simulink model "Modellering"  (R2026a)
settings: Solver=VariableStepAuto  StopTime=24*T_time  AbsTol=1e-3
values from neighbouring files (symbols this model uses):
  E_batt_Wh = 1e3    (= 1000)    [Solcelle_KW_PR_KWP.m]
  pf_fabrik = 0.85    [Last_fra_fabrik_blokkode.m]
  T_time = 0.2    [Solcelle_KW_PR_KWP.m]
libraries: ee_lib x24, nesl_utility x23, eeSinGeneratorThreePhase x3, fl_lib x2
settings Model: Creator=Tjalf  LastModifiedBy=Tjalf
settings DebuggingCC: SymbolicDimsDataTypeCodeGenerationDiagnostic=none

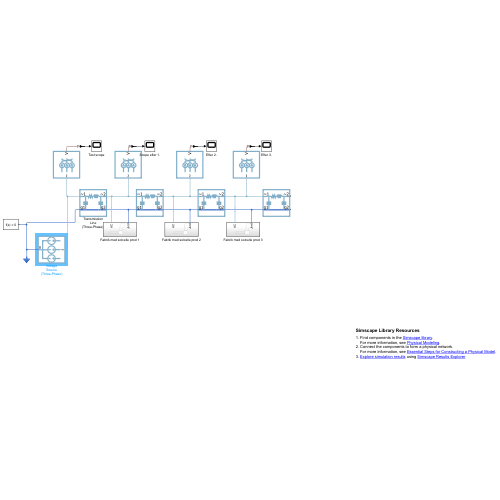
[thumbnail: Simulink's stored preview of the top-level diagram]
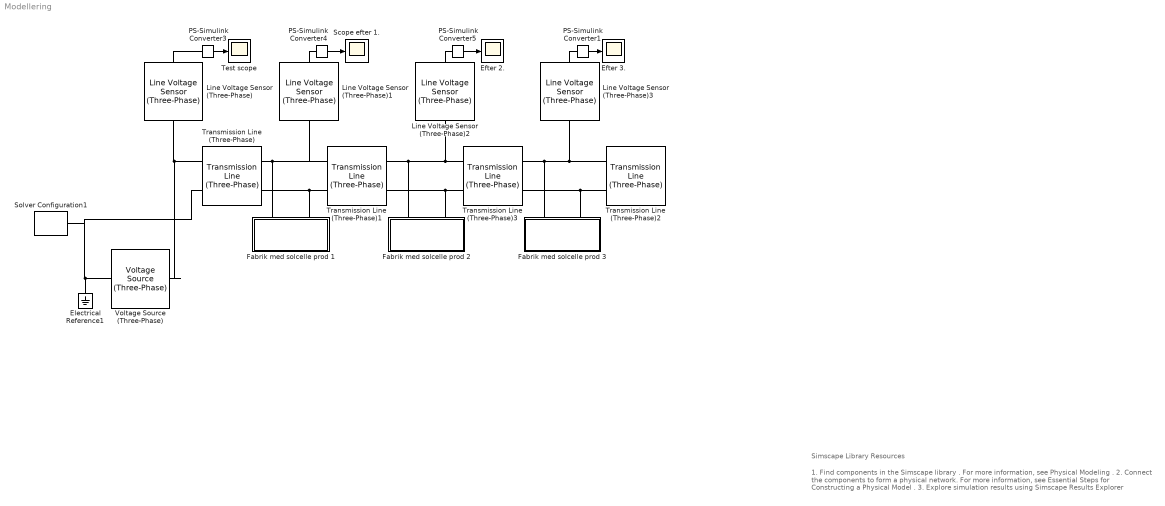
== system Modellering ==
  note: 1. Find components in the Simscape library .
      | For more information, see Physical Modeling .
      | 2. Connect the components to form a physical network.
      | For more information, see Essential Steps for Constructing a Physical Model .
      | 3. Explore simulation results using Simscape Results Explorer
  note: Simscape Library Resources
  Efter 2. : Scope
      settings: ActiveDisplayYMinimum=-525.7657436259899  ActiveDisplayYMaximum=512.09070122953233  DataLoggingVariableName=ScopeData5
  Efter 3. : Scope
      settings: ActiveDisplayYMinimum=-108.97469280207605  ActiveDisplayYMaximum=205.85166313411651  DataLoggingVariableName=ScopeData2
  Electrical Reference1 : fl_lib/Electrical/Electrical Elements/Electrical Reference
  Fabrik med solcelle prod 1 : Subsystem
      settings: PortSchema="{\"entries\":[{\"content\":{\"sides\":[{\"content\":{},\"type\":\"ConnectorPlacement.EquallySpacedRectSide\",\"uuid\":\"8903bc28-abed-4d25-a485-866d339a2aaa\"},{\"content\":{\"side\":\"RIGHT\"},\"type\":\"ConnectorPlacement.EquallySpacedRectSide\",\"uuid\":\"5b54d37e-ff1f-4c27-bd8c-71a5161d98d9\"},{\"content\":{\"connectorIds\":[\"LConn1\",\"LConn2\"],\"side\":\"TOP\"},\"type\":\"ConnectorPlacement.EquallySpacedRectSide\",\"uuid\":\"1a79fc57-00bb-46c3-a083-8bac977ee0cf\"},{\"content\":{\"side\":\"BOTTOM\"},\"type\":\"ConnectorPlacement.EquallySpacedRectSide\",\"uuid\":\"fed7dcc3-d9d7-4755-8d81-a67162f2978b\"}]},\"type\":\"ConnectorPlacement.EquallySpacedConnector\",\"uuid\":\"4f69986a-bdbb-438c-8339-f1c9bb70dacd\"}],\"packageUris\":[\"http://schema.mathworks.com/mf0/Connector/R2020b\"],\"version\":\"1.0\"}"
  Fabrik med solcelle prod 2 : Subsystem
      settings: PortSchema="{\"entries\":[{\"content\":{\"sides\":[{\"content\":{},\"type\":\"ConnectorPlacement.EquallySpacedRectSide\",\"uuid\":\"8903bc28-abed-4d25-a485-866d339a2aaa\"},{\"content\":{\"side\":\"RIGHT\"},\"type\":\"ConnectorPlacement.EquallySpacedRectSide\",\"uuid\":\"5b54d37e-ff1f-4c27-bd8c-71a5161d98d9\"},{\"content\":{\"connectorIds\":[\"LConn1\",\"LConn2\"],\"side\":\"TOP\"},\"type\":\"ConnectorPlacement.EquallySpacedRectSide\",\"uuid\":\"1a79fc57-00bb-46c3-a083-8bac977ee0cf\"},{\"content\":{\"side\":\"BOTTOM\"},\"type\":\"ConnectorPlacement.EquallySpacedRectSide\",\"uuid\":\"fed7dcc3-d9d7-4755-8d81-a67162f2978b\"}]},\"type\":\"ConnectorPlacement.EquallySpacedConnector\",\"uuid\":\"4f69986a-bdbb-438c-8339-f1c9bb70dacd\"}],\"packageUris\":[\"http://schema.mathworks.com/mf0/Connector/R2020b\"],\"version\":\"1.0\"}"
  Fabrik med solcelle prod 3 : Subsystem
      settings: PortSchema="{\"entries\":[{\"content\":{\"sides\":[{\"content\":{},\"type\":\"ConnectorPlacement.EquallySpacedRectSide\",\"uuid\":\"8903bc28-abed-4d25-a485-866d339a2aaa\"},{\"content\":{\"side\":\"RIGHT\"},\"type\":\"ConnectorPlacement.EquallySpacedRectSide\",\"uuid\":\"5b54d37e-ff1f-4c27-bd8c-71a5161d98d9\"},{\"content\":{\"connectorIds\":[\"LConn1\",\"LConn2\"],\"side\":\"TOP\"},\"type\":\"ConnectorPlacement.EquallySpacedRectSide\",\"uuid\":\"1a79fc57-00bb-46c3-a083-8bac977ee0cf\"},{\"content\":{\"side\":\"BOTTOM\"},\"type\":\"ConnectorPlacement.EquallySpacedRectSide\",\"uuid\":\"fed7dcc3-d9d7-4755-8d81-a67162f2978b\"}]},\"type\":\"ConnectorPlacement.EquallySpacedConnector\",\"uuid\":\"4f69986a-bdbb-438c-8339-f1c9bb70dacd\"}],\"packageUris\":[\"http://schema.mathworks.com/mf0/Connector/R2020b\"],\"version\":\"1.0\"}"
  Line Voltage Sensor (Three-Phase){,1..3} (4 alike) : ee_lib/Sensors & Transducers/Line Voltage Sensor (Three-Phase)  port_option=ee.enum.threePhasePort.composite
  PS-Simulink Converter{1,3..5} (4 alike) : nesl_utility/PS-Simulink Converter  PhysicalDomain=network_engine_domain  SubClassName=ps_output  LeftPortType=input  RightPortType=output  PseudoPeriodic=off  Frequencies=[]  VectorFormat=inherit  Unit=V  AffineConversion=off
  Scope efter 1. : Scope
      settings: ActiveDisplayYMinimum=-808.59258984260134  ActiveDisplayYMaximum=1226.7327895966071  DataLoggingVariableName=ScopeData4
  Solver Configuration1 : nesl_utility/Solver Configuration  PhysicalDomain=network_engine_domain  SubClassName=solver  LeftPortType=input  RightPortType=generic  Tones=[]  Harmonics=[]  SimulateNoise=off  Profile=off  UseLocalSampling=off  EnableSwitchedLinearOptims=on  FrequencyDomain=off  UseCCode=off  RelTol=0.001  AbsTol=0.001  MinStep=1e-09  ToWorkspace=off  RevertToSquareIcSolve=off  NumHomotopyIterations=100  PhasorMode=off  PhasorModeNumHarmonics=1  ConsistencySolver=NEWTON_XTOL_AFTER_FTOL  CanonicalOrdering=CANONICAL  OptimizeIntermediates=OPTIMIZED  IndexReductionMethod=DerivativeReplacement  DoDC=off  ResidualTolerance=1e-09  ConsistencyTolSource=GLOBAL  ConsistencyAbsTol=0.001  ConsistencyRelTol=0.001  ConsistencyTolFactor=0.001  UseLocalSolver=on  LocalSolverChoice=NE_BACKWARD_EULER_ADVANCER  ResolveIndetEquations=on  FunctionEvalNumThread=1  LocalSolverSampleTime=1e-4  DoFixedCost=off  MaxNonlinIter=3  MaxModeIter=2  ComputeImpulses=off  ImpulseIterations=2  LinearAlgebra=auto  LinearAlgebraNumThread=0  EquationFormulation=NE_TIME_EF  DelaysMemoryBudget=1024  AutomaticFiltering=on  FilteringTimeConstant=0.001  PartitionStorageMethod=AS_NEEDED  PartitionMemoryBudget=1024  PartitionMethod=ROBUST  MultibodyUseLocalSolver=off  MultibodyLocalSolverChoice=ODE1  MultibodyLocalSolverSampleTime=0.001
  Test scope : Scope
      settings: ActiveDisplayYMinimum=-725.330758823431  ActiveDisplayYMaximum=222.55952159059962  DataLoggingVariableName=ScopeData3
  "Transmission Line (Three-Phase) " : ee_lib/Passive/Lines/Transmission Line (Three-Phase)  port_option=ee.enum.threePhasePort.composite  length=0.4 km  freq=50 Hz  prm=ee.enum.lines.parameterization3ph.physicalLineParam  R=0.34 Ohm/km  Rm=0 Ohm/km  L=0.5 mH/km  M=0.1 mH/km  Cl=0.3 uF/km  Cg=0.1 uF/km  Rpos=0.01 Ohm/km  Rzero=0.04 Ohm/km  Lpos=0.4 mH/km  Lzero=0.7 mH/km  Cpos=1 uF/km  Czero=0.1 uF/km  ModelTwoSections=ee.enum.enable.no  N=1  InterfacePosition=0.5 km  N1sec=1  N2sec=1  Access_ground=ee.enum.enable.no  R_parasitic=1e-6 Ohm  G_parasitic=1e-6 1/Ohm
  Transmission Line (Three-Phase)1 : ee_lib/Passive/Lines/Transmission Line (Three-Phase)  port_option=ee.enum.threePhasePort.composite  length=0.2 km  freq=50 Hz  prm=ee.enum.lines.parameterization3ph.physicalLineParam  R=0.34 Ohm/km  Rm=0 Ohm/km  L=0.5 mH/km  M=0.1 mH/km  Cl=0.3 uF/km  Cg=0.1 uF/km  Rpos=0.01 Ohm/km  Rzero=0.04 Ohm/km  Lpos=0.4 mH/km  Lzero=0.7 mH/km  Cpos=1 uF/km  Czero=0.1 uF/km  ModelTwoSections=ee.enum.enable.no  N=1  InterfacePosition=0.5 km  N1sec=1  N2sec=1  Access_ground=ee.enum.enable.no  R_parasitic=1e-6 Ohm  G_parasitic=1e-6 1/Ohm
  Transmission Line (Three-Phase)2 : ee_lib/Passive/Lines/Transmission Line (Three-Phase)  port_option=ee.enum.threePhasePort.composite  length=0.3 km  freq=50 Hz  prm=ee.enum.lines.parameterization3ph.physicalLineParam  R=0.34 Ohm/km  Rm=0 Ohm/km  L=0.5 mH/km  M=0.1 mH/km  Cl=0.3 uF/km  Cg=0.1 uF/km  Rpos=0.01 Ohm/km  Rzero=0.04 Ohm/km  Lpos=0.4 mH/km  Lzero=0.7 mH/km  Cpos=1 uF/km  Czero=0.1 uF/km  ModelTwoSections=ee.enum.enable.no  N=1  InterfacePosition=0.5 km  N1sec=1  N2sec=1  Access_ground=ee.enum.enable.no  R_parasitic=1e-6 Ohm  G_parasitic=1e-6 1/Ohm
  Transmission Line (Three-Phase)3 : ee_lib/Passive/Lines/Transmission Line (Three-Phase)  port_option=ee.enum.threePhasePort.composite  length=0.3 km  freq=50 Hz  prm=ee.enum.lines.parameterization3ph.physicalLineParam  R=0.34 Ohm/km  Rm=0 Ohm/km  L=0.5 mH/km  M=0.1 mH/km  Cl=0.3 uF/km  Cg=0.1 uF/km  Rpos=0.01 Ohm/km  Rzero=0.04 Ohm/km  Lpos=0.4 mH/km  Lzero=0.7 mH/km  Cpos=1 uF/km  Czero=0.1 uF/km  ModelTwoSections=ee.enum.enable.no  N=1  InterfacePosition=0.5 km  N1sec=1  N2sec=1  Access_ground=ee.enum.enable.no  R_parasitic=1e-6 Ohm  G_parasitic=1e-6 1/Ohm
  Voltage Source (Three-Phase) : ee_lib/Sources/Voltage Source (Three-Phase)  vline_rms=400 V  shift=0 deg  freq=50 Hz  impedance_option=1  SShortCircuit=1e9 A*V  XR=15  R=0.01 Ohm  L=3.97e-4 H  harmonic_option=0  harmonic_orders=[5, 7, 11, 13]  harmonic_ratios=[.1, .1, .1, .1]  G_parasitic=0 1/Ohm  I_specify=off  I_priority=None  I=[0, 0, 0] A  I_nominal_specify=off  I_nominal_value=1  I_nominal_unit=A
  wires:
  PS-Simulink Converter3/1 -> Test scope/1
  PS-Simulink Converter4/1 -> Scope efter 1./1
  PS-Simulink Converter5/1 -> Efter 2./1
  PS-Simulink Converter1/1 -> Efter 3./1
  connections:
  Electrical Reference1/LConn1 -- "Transmission Line (Three-Phase) "/LConn2 -- Solver Configuration1/RConn1 -- Voltage Source (Three-Phase)/LConn1
  Voltage Source (Three-Phase)/RConn1 -- Line Voltage Sensor (Three-Phase)/LConn1 -- "Transmission Line (Three-Phase) "/LConn1
  Transmission Line (Three-Phase)3/LConn1 -- Fabrik med solcelle prod 2/LConn1 -- Transmission Line (Three-Phase)1/RConn1 -- Line Voltage Sensor (Three-Phase)2/LConn1
  Transmission Line (Three-Phase)3/LConn2 -- Fabrik med solcelle prod 2/LConn2 -- Transmission Line (Three-Phase)1/RConn2
  Transmission Line (Three-Phase)1/LConn2 -- Fabrik med solcelle prod 1/LConn2 -- "Transmission Line (Three-Phase) "/RConn2
  "Transmission Line (Three-Phase) "/RConn1 -- Transmission Line (Three-Phase)1/LConn1 -- Line Voltage Sensor (Three-Phase)1/LConn1 -- Fabrik med solcelle prod 1/LConn1
  Line Voltage Sensor (Three-Phase)/RConn1 -- PS-Simulink Converter3/LConn1
  Line Voltage Sensor (Three-Phase)1/RConn1 -- PS-Simulink Converter4/LConn1
  Line Voltage Sensor (Three-Phase)2/RConn1 -- PS-Simulink Converter5/LConn1
  Line Voltage Sensor (Three-Phase)3/RConn1 -- PS-Simulink Converter1/LConn1
  Line Voltage Sensor (Three-Phase)3/LConn1 -- Fabrik med solcelle prod 3/LConn1 -- Transmission Line (Three-Phase)3/RConn1 -- Transmission Line (Three-Phase)2/LConn1
  Transmission Line (Three-Phase)2/LConn2 -- Fabrik med solcelle prod 3/LConn2 -- Transmission Line (Three-Phase)3/RConn2

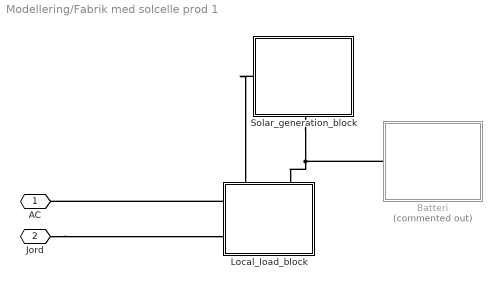
== system Modellering/Fabrik med solcelle prod 1 ==
  Batteri : Subsystem  Commented=on
  Local_load_block : Subsystem
      settings: PortSchema="{\"entries\":[{\"content\":{\"sides\":[{\"content\":{\"connectorIds\":[\"LConn1\",\"LConn2\"]},\"type\":\"ConnectorPlacement.EquallySpacedRectSide\",\"uuid\":\"b9fbc9ff-ac4f-4b90-979a-9a6eda85b56b\"},{\"content\":{\"side\":\"RIGHT\"},\"type\":\"ConnectorPlacement.EquallySpacedRectSide\",\"uuid\":\"0bc181a9-ce47-4155-858d-d096cf0eda13\"},{\"content\":{\"connectorIds\":[\"LConn3\",\"LConn4\"],\"side\":\"TOP\"},\"type\":\"ConnectorPlacement.EquallySpacedRectSide\",\"uuid\":\"c62c2ae1-dcbf-4404-92e0-79f349a5ed39\"}]},\"type\":\"ConnectorPlacement.EquallySpacedConnector\",\"uuid\":\"35e445ba-d9d4-4891-abed-fc367708c4b2\"}],\"packageUris\":[\"http://schema.mathworks.com/mf0/Connector/R2020b\"],\"version\":\"1.0\"}"
  Solar_generation_block : Subsystem
      settings: PortSchema="{\"entries\":[{\"content\":{\"sides\":[{\"content\":{\"connectorIds\":[\"LConn1\"]},\"type\":\"ConnectorPlacement.EquallySpacedRectSide\",\"uuid\":\"cbc424fc-8eab-49e5-bd35-99b901f58cde\"},{\"content\":{\"side\":\"RIGHT\"},\"type\":\"ConnectorPlacement.EquallySpacedRectSide\",\"uuid\":\"42c77621-fd98-407f-9927-3f3ead5ecc38\"},{\"content\":{\"side\":\"TOP\"},\"type\":\"ConnectorPlacement.EquallySpacedRectSide\",\"uuid\":\"f218016a-264e-4591-beac-7ee07d8c289f\"},{\"content\":{\"connectorIds\":[\"RConn1\"],\"side\":\"BOTTOM\"},\"type\":\"ConnectorPlacement.EquallySpacedRectSide\",\"uuid\":\"65d2543d-d490-4083-b53c-51918d15ba9f\"}]},\"type\":\"ConnectorPlacement.EquallySpacedConnector\",\"uuid\":\"55afaa4f-6643-4b7e-8511-738cdc79d4c6\"}],\"packageUris\":[\"http://schema.mathworks.com/mf0/Connector/R2020b\"],\"version\":\"1.0\"}"
  AC : PMIOPort  Side=Left
  Jord : PMIOPort  Port=2  Side=Left
  connections:
  Local_load_block/LConn1 -- AC/RConn1
  Jord/RConn1 -- Local_load_block/LConn2
  Solar_generation_block/LConn1 -- Local_load_block/LConn3
  Solar_generation_block/RConn1 -- Batteri/LConn1 -- Local_load_block/LConn4

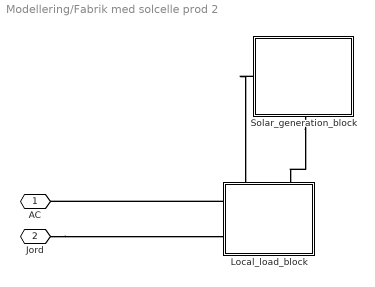
== system Modellering/Fabrik med solcelle prod 2 ==
  Local_load_block : Subsystem
      settings: PortSchema="{\"entries\":[{\"content\":{\"sides\":[{\"content\":{\"connectorIds\":[\"LConn1\",\"LConn2\"]},\"type\":\"ConnectorPlacement.EquallySpacedRectSide\",\"uuid\":\"b9fbc9ff-ac4f-4b90-979a-9a6eda85b56b\"},{\"content\":{\"side\":\"RIGHT\"},\"type\":\"ConnectorPlacement.EquallySpacedRectSide\",\"uuid\":\"0bc181a9-ce47-4155-858d-d096cf0eda13\"},{\"content\":{\"connectorIds\":[\"LConn3\",\"LConn4\"],\"side\":\"TOP\"},\"type\":\"ConnectorPlacement.EquallySpacedRectSide\",\"uuid\":\"c62c2ae1-dcbf-4404-92e0-79f349a5ed39\"}]},\"type\":\"ConnectorPlacement.EquallySpacedConnector\",\"uuid\":\"35e445ba-d9d4-4891-abed-fc367708c4b2\"}],\"packageUris\":[\"http://schema.mathworks.com/mf0/Connector/R2020b\"],\"version\":\"1.0\"}"
  Solar_generation_block : Subsystem
      settings: PortSchema="{\"entries\":[{\"content\":{\"sides\":[{\"content\":{\"connectorIds\":[\"LConn1\"]},\"type\":\"ConnectorPlacement.EquallySpacedRectSide\",\"uuid\":\"cbc424fc-8eab-49e5-bd35-99b901f58cde\"},{\"content\":{\"side\":\"RIGHT\"},\"type\":\"ConnectorPlacement.EquallySpacedRectSide\",\"uuid\":\"42c77621-fd98-407f-9927-3f3ead5ecc38\"},{\"content\":{\"side\":\"TOP\"},\"type\":\"ConnectorPlacement.EquallySpacedRectSide\",\"uuid\":\"f218016a-264e-4591-beac-7ee07d8c289f\"},{\"content\":{\"connectorIds\":[\"RConn1\"],\"side\":\"BOTTOM\"},\"type\":\"ConnectorPlacement.EquallySpacedRectSide\",\"uuid\":\"65d2543d-d490-4083-b53c-51918d15ba9f\"}]},\"type\":\"ConnectorPlacement.EquallySpacedConnector\",\"uuid\":\"55afaa4f-6643-4b7e-8511-738cdc79d4c6\"}],\"packageUris\":[\"http://schema.mathworks.com/mf0/Connector/R2020b\"],\"version\":\"1.0\"}"
  AC : PMIOPort  Side=Left
  Jord : PMIOPort  Port=2  Side=Left
  connections:
  Solar_generation_block/RConn1 -- Local_load_block/LConn4
  Solar_generation_block/LConn1 -- Local_load_block/LConn3
  Jord/RConn1 -- Local_load_block/LConn2
  Local_load_block/LConn1 -- AC/RConn1

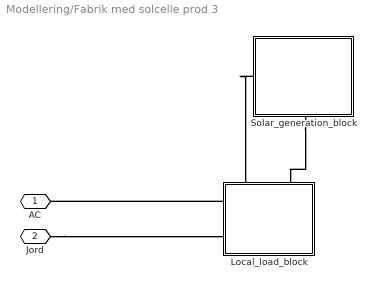
== system Modellering/Fabrik med solcelle prod 3 ==
  Local_load_block : Subsystem
      settings: PortSchema="{\"entries\":[{\"content\":{\"sides\":[{\"content\":{\"connectorIds\":[\"LConn1\",\"LConn2\"]},\"type\":\"ConnectorPlacement.EquallySpacedRectSide\",\"uuid\":\"b9fbc9ff-ac4f-4b90-979a-9a6eda85b56b\"},{\"content\":{\"side\":\"RIGHT\"},\"type\":\"ConnectorPlacement.EquallySpacedRectSide\",\"uuid\":\"0bc181a9-ce47-4155-858d-d096cf0eda13\"},{\"content\":{\"connectorIds\":[\"LConn3\",\"LConn4\"],\"side\":\"TOP\"},\"type\":\"ConnectorPlacement.EquallySpacedRectSide\",\"uuid\":\"c62c2ae1-dcbf-4404-92e0-79f349a5ed39\"}]},\"type\":\"ConnectorPlacement.EquallySpacedConnector\",\"uuid\":\"35e445ba-d9d4-4891-abed-fc367708c4b2\"}],\"packageUris\":[\"http://schema.mathworks.com/mf0/Connector/R2020b\"],\"version\":\"1.0\"}"
  Solar_generation_block : Subsystem
      settings: PortSchema="{\"entries\":[{\"content\":{\"sides\":[{\"content\":{\"connectorIds\":[\"LConn1\"]},\"type\":\"ConnectorPlacement.EquallySpacedRectSide\",\"uuid\":\"cbc424fc-8eab-49e5-bd35-99b901f58cde\"},{\"content\":{\"side\":\"RIGHT\"},\"type\":\"ConnectorPlacement.EquallySpacedRectSide\",\"uuid\":\"42c77621-fd98-407f-9927-3f3ead5ecc38\"},{\"content\":{\"side\":\"TOP\"},\"type\":\"ConnectorPlacement.EquallySpacedRectSide\",\"uuid\":\"f218016a-264e-4591-beac-7ee07d8c289f\"},{\"content\":{\"connectorIds\":[\"RConn1\"],\"side\":\"BOTTOM\"},\"type\":\"ConnectorPlacement.EquallySpacedRectSide\",\"uuid\":\"65d2543d-d490-4083-b53c-51918d15ba9f\"}]},\"type\":\"ConnectorPlacement.EquallySpacedConnector\",\"uuid\":\"55afaa4f-6643-4b7e-8511-738cdc79d4c6\"}],\"packageUris\":[\"http://schema.mathworks.com/mf0/Connector/R2020b\"],\"version\":\"1.0\"}"
  AC : PMIOPort  Side=Left
  Jord : PMIOPort  Port=2  Side=Left
  connections:
  Solar_generation_block/RConn1 -- Local_load_block/LConn4
  Solar_generation_block/LConn1 -- Local_load_block/LConn3
  Jord/RConn1 -- Local_load_block/LConn2
  Local_load_block/LConn1 -- AC/RConn1

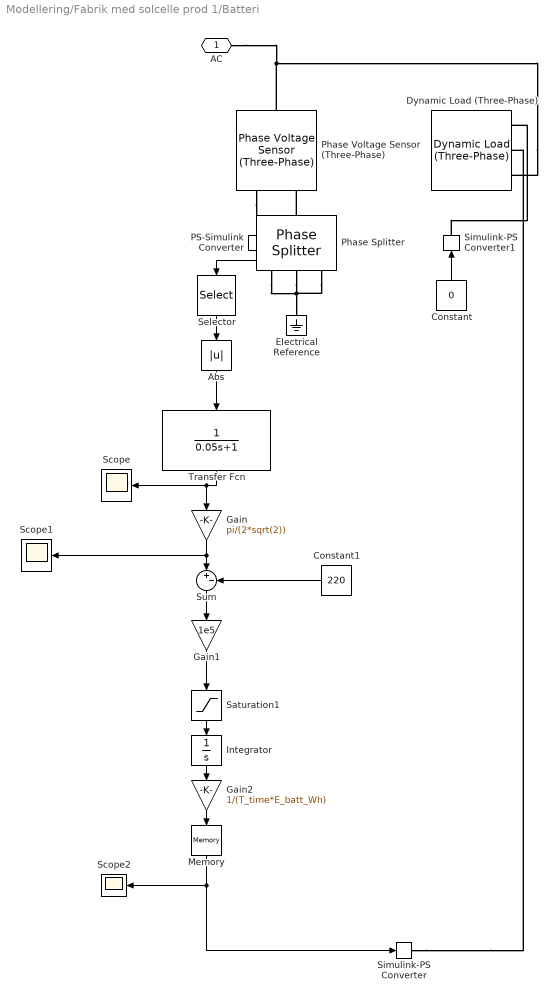
== system Modellering/Fabrik med solcelle prod 1/Batteri ==
  Abs : Abs  SaturateOnIntegerOverflow=off
  Constant : Constant  Value=0
  Constant1 : Constant  Value=220
  Dynamic Load (Three-Phase) : ee_lib/Passive/Dynamic Load (Three-Phase)  port_option=ee.enum.threePhasePort.composite  FRated=60 Hz  Vline_rms_min=100 V  tau=0.01 s  Vline_rms_ini=200 V  Vang_ini=0 deg  gmin=0 S
  Electrical Reference : fl_lib/Electrical/Electrical Elements/Electrical Reference
  Gain : Gain  Gain=pi/(2*sqrt(2))
  Gain1 : Gain  Gain=1e5
  Gain2 : Gain  Gain=1/(T_time*E_batt_Wh)
  Integrator : Integrator
  Memory : Memory
  PS-Simulink Converter : nesl_utility/PS-Simulink Converter  PhysicalDomain=network_engine_domain  SubClassName=ps_output  LeftPortType=input  RightPortType=output  PseudoPeriodic=off  Frequencies=[]  VectorFormat=inherit  Unit=inherit  AffineConversion=off
  Phase Splitter : ee_lib/Connectors & References/Phase Splitter
  Phase Voltage Sensor (Three-Phase) : ee_lib/Sensors & Transducers/Phase Voltage Sensor (Three-Phase)  port_option=ee.enum.threePhasePort.composite
  Saturation1 : Saturate  UpperLimit=500e3  LowerLimit=0
  Scope : Scope
      settings: ActiveDisplayYMinimum=-188.85965890115085  ActiveDisplayYMaximum=455.68910443657887  DataLoggingVariableName=ScopeData6
  Scope1 : Scope
      settings: ActiveDisplayYMinimum=-209.2949841576883  ActiveDisplayYMaximum=444.97038901782815  DataLoggingVariableName=ScopeData7
  Scope2 : Scope
      settings: ActiveDisplayYMinimum=-609.68485948765465  ActiveDisplayYMaximum=719.66818650943037  DataLoggingVariableName=ScopeData8
  Selector : Selector  InputPortWidth=3  IndexOptions=Index vector (dialog)  Indices=[1]  OutputSizes=1
  Simulink-PS Converter : nesl_utility/Simulink-PS Converter  PhysicalDomain=network_engine_domain  SubClassName=ps_input  LeftPortType=input  RightPortType=output  PseudoPeriodic=off  Frequencies=[]  NoiseDistribution=none  NoiseParameters=[]  Unit=1  AffineConversion=off  FilteringAndDerivatives=provide  SimscapeFilterOrder=1  InputFilterTimeConstant=0.001  UdotUserProvided=0
  Simulink-PS Converter1 : nesl_utility/Simulink-PS Converter  PhysicalDomain=network_engine_domain  SubClassName=ps_input  LeftPortType=input  RightPortType=output  PseudoPeriodic=off  Frequencies=[]  NoiseDistribution=none  NoiseParameters=[]  Unit=1  AffineConversion=off  FilteringAndDerivatives=provide  SimscapeFilterOrder=1  InputFilterTimeConstant=0.001  UdotUserProvided=0
  Sum : Sum  Inputs=|+-
  Transfer Fcn : TransferFcn  Denominator=[0.05 1]
  AC : PMIOPort  Side=Left
  wires:
  PS-Simulink Converter/1 -> Selector/1
  Selector/1 -> Abs/1
  Abs/1 -> Transfer Fcn/1
  Transfer Fcn/1 -> Scope/1, Gain/1
  Constant/1 -> Simulink-PS Converter1/1
  Gain/1 -> Scope1/1, Sum/1
  Constant1/1 -> Sum/2
  Sum/1 -> Gain1/1
  Gain1/1 -> Saturation1/1
  Memory/1 -> Simulink-PS Converter/1, Scope2/1
  Saturation1/1 -> Integrator/1
  Integrator/1 -> Gain2/1
  Gain2/1 -> Memory/1
  connections:
  AC/RConn1 -- Phase Voltage Sensor (Three-Phase)/LConn1 -- Dynamic Load (Three-Phase)/LConn1
  Phase Splitter/LConn1 -- Phase Voltage Sensor (Three-Phase)/RConn2
  Phase Splitter/RConn3 -- Phase Splitter/RConn1 -- Electrical Reference/LConn1 -- Phase Splitter/RConn2
  Phase Voltage Sensor (Three-Phase)/RConn1 -- PS-Simulink Converter/LConn1
  Simulink-PS Converter/RConn1 -- Dynamic Load (Three-Phase)/LConn2
  Simulink-PS Converter1/RConn1 -- Dynamic Load (Three-Phase)/LConn3

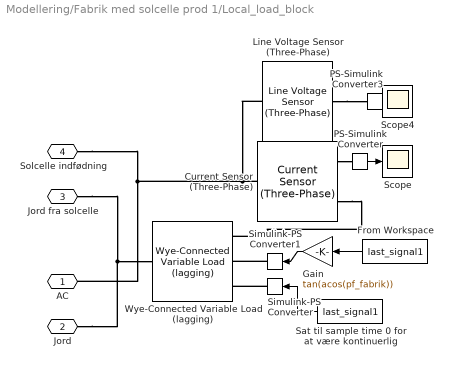
== system Modellering/Fabrik med solcelle prod 1/Local_load_block ==
  Current Sensor (Three-Phase) : ee_lib/Sensors & Transducers/Current Sensor (Three-Phase)  port_option=ee.enum.threePhasePort.composite
  From Workspace : FromWorkspace  VariableName=last_signal1
  Gain : Gain  Gain=tan(acos(pf_fabrik))
  Line Voltage Sensor (Three-Phase) : ee_lib/Sensors & Transducers/Line Voltage Sensor (Three-Phase)  port_option=ee.enum.threePhasePort.composite
  PS-Simulink Converter : nesl_utility/PS-Simulink Converter  PhysicalDomain=network_engine_domain  SubClassName=ps_output  LeftPortType=input  RightPortType=output  PseudoPeriodic=off  Frequencies=[]  VectorFormat=inherit  Unit=A  AffineConversion=off
  PS-Simulink Converter3 : nesl_utility/PS-Simulink Converter  PhysicalDomain=network_engine_domain  SubClassName=ps_output  LeftPortType=input  RightPortType=output  PseudoPeriodic=off  Frequencies=[]  VectorFormat=inherit  Unit=V  AffineConversion=off
  Sat til sample time 0 for at være kontinuerlig : FromWorkspace  VariableName=last_signal1  Interpolate=off  OutputAfterFinalValue=Holding final value
  Scope : Scope
      settings: ActiveDisplayYMinimum=-321.52156371284451  ActiveDisplayYMaximum=409.38065684966335
  Scope4 : Scope
      settings: ActiveDisplayYMinimum=-724.32967100373537  ActiveDisplayYMaximum=544.90361596398475
  Simulink-PS Converter : nesl_utility/Simulink-PS Converter  PhysicalDomain=network_engine_domain  SubClassName=ps_input  LeftPortType=input  RightPortType=output  PseudoPeriodic=off  Frequencies=[]  NoiseDistribution=none  NoiseParameters=[]  Unit=1  AffineConversion=off  FilteringAndDerivatives=provide  SimscapeFilterOrder=1  InputFilterTimeConstant=0.001  UdotUserProvided=0
  Simulink-PS Converter1 : nesl_utility/Simulink-PS Converter  PhysicalDomain=network_engine_domain  SubClassName=ps_input  LeftPortType=input  RightPortType=output  PseudoPeriodic=off  Frequencies=[]  NoiseDistribution=none  NoiseParameters=[]  Unit=1  AffineConversion=off  FilteringAndDerivatives=provide  SimscapeFilterOrder=1  InputFilterTimeConstant=0.001  UdotUserProvided=0
  "Wye-Connected Variable Load (lagging) " : ee_lib/Passive/RLC Assemblies/Wye-Connected Variable Load (lagging)  port_option=ee.enum.threePhasePort.composite  VRated=400 V  FRated=50 Hz  Pmin=1e3 W  Qmin=1e3 A*V  G_parasitic=1e-6 1/Ohm  I_specify=off  I_priority=None  I=[0, 0, 0] A  I_nominal_specify=off  I_nominal_value=1  I_nominal_unit=A  Phi_specify=off  Phi_priority=None  Phi=[0, 0, 0] Wb  Phi_nominal_specify=off  Phi_nominal_value=1  Phi_nominal_unit=Wb
  AC : PMIOPort  Side=Left
  Jord : PMIOPort  Port=2  Side=Left
  Jord fra solcelle : PMIOPort  Port=3  Side=Left
  Solcelle indfødning : PMIOPort  Port=4  Side=Left
  wires:
  PS-Simulink Converter3/1 -> Scope4/1
  PS-Simulink Converter/1 -> Scope/1
  Sat til sample time 0 for at være kontinuerlig/1 -> Simulink-PS Converter/1
  From Workspace/1 -> Gain/1
  Gain/1 -> Simulink-PS Converter1/1
  connections:
  Current Sensor (Three-Phase)/RConn2 -- "Wye-Connected Variable Load (lagging) "/LConn3
  Current Sensor (Three-Phase)/LConn1 -- AC/RConn1 -- Solcelle indfødning/RConn1 -- Line Voltage Sensor (Three-Phase)/LConn1
  Jord/RConn1 -- Jord fra solcelle/RConn1 -- "Wye-Connected Variable Load (lagging) "/RConn1
  Line Voltage Sensor (Three-Phase)/RConn1 -- PS-Simulink Converter3/LConn1
  Current Sensor (Three-Phase)/RConn1 -- PS-Simulink Converter/LConn1
  Simulink-PS Converter/RConn1 -- "Wye-Connected Variable Load (lagging) "/LConn1
  Simulink-PS Converter1/RConn1 -- "Wye-Connected Variable Load (lagging) "/LConn2

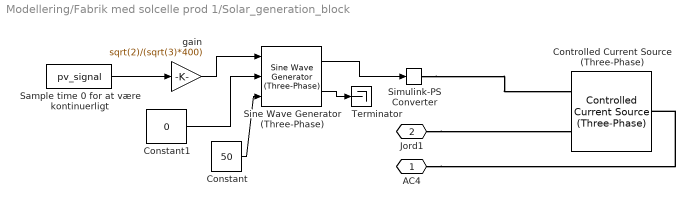
== system Modellering/Fabrik med solcelle prod 1/Solar_generation_block ==
  Constant : Constant  Value=50
  Constant1 : Constant  Value=0
  Controlled Current Source (Three-Phase) : ee_lib/Sources/Controlled Current Source (Three-Phase)  port_option=ee.enum.threePhasePort.composite  input_option=ee.enum.inputType.instantaneous  FRated=60 Hz  G_parasitic=1e-6 1/Ohm
  Sample time 0 for at være kontinuerligt : FromWorkspace  VariableName=pv_signal  Interpolate=off  OutputAfterFinalValue=Holding final value
  Simulink-PS Converter : nesl_utility/Simulink-PS Converter  PhysicalDomain=network_engine_domain  SubClassName=ps_input  LeftPortType=input  RightPortType=output  PseudoPeriodic=off  Frequencies=[]  NoiseDistribution=none  NoiseParameters=[]  Unit=1  AffineConversion=off  FilteringAndDerivatives=provide  SimscapeFilterOrder=1  InputFilterTimeConstant=0.001  UdotUserProvided=0
  Sine Wave Generator (Three-Phase) : eeSinGeneratorThreePhase/Sine Wave Generator (Three-Phase)  Ts=0
      settings: LibrarySourceBlock=|
      | ee_sl_lib/General Control/Sine Wave Generator
      | (Three-Phase)
  Terminator : Terminator
  gain : Gain  Gain=sqrt(2)/(sqrt(3)*400)
  AC4 : PMIOPort  Side=Right
  Jord1 : PMIOPort  Port=2  Side=Left
  wires:
  Sample time 0 for at være kontinuerligt/1 -> gain/1
  Constant/1 -> Sine Wave Generator (Three-Phase)/3
  Constant1/1 -> Sine Wave Generator (Three-Phase)/2
  gain/1 -> Sine Wave Generator (Three-Phase)/1
  Sine Wave Generator (Three-Phase)/1 -> Simulink-PS Converter/1
  Sine Wave Generator (Three-Phase)/2 -> Terminator/1
  connections:
  AC4/RConn1 -- Controlled Current Source (Three-Phase)/RConn1
  Jord1/RConn1 -- Controlled Current Source (Three-Phase)/LConn2
  Simulink-PS Converter/RConn1 -- Controlled Current Source (Three-Phase)/LConn1

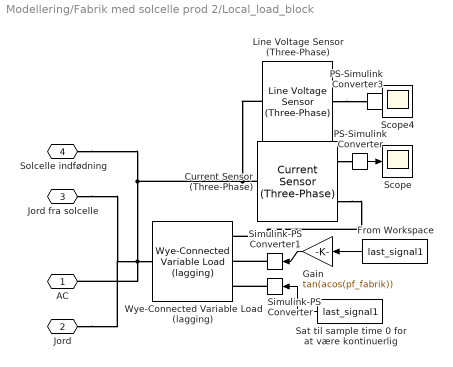
== system Modellering/Fabrik med solcelle prod 2/Local_load_block ==
  Current Sensor (Three-Phase) : ee_lib/Sensors & Transducers/Current Sensor (Three-Phase)  port_option=ee.enum.threePhasePort.composite
  From Workspace : FromWorkspace  VariableName=last_signal1
  Gain : Gain  Gain=tan(acos(pf_fabrik))
  Line Voltage Sensor (Three-Phase) : ee_lib/Sensors & Transducers/Line Voltage Sensor (Three-Phase)  port_option=ee.enum.threePhasePort.composite
  PS-Simulink Converter : nesl_utility/PS-Simulink Converter  PhysicalDomain=network_engine_domain  SubClassName=ps_output  LeftPortType=input  RightPortType=output  PseudoPeriodic=off  Frequencies=[]  VectorFormat=inherit  Unit=A  AffineConversion=off
  PS-Simulink Converter3 : nesl_utility/PS-Simulink Converter  PhysicalDomain=network_engine_domain  SubClassName=ps_output  LeftPortType=input  RightPortType=output  PseudoPeriodic=off  Frequencies=[]  VectorFormat=inherit  Unit=V  AffineConversion=off
  Sat til sample time 0 for at være kontinuerlig : FromWorkspace  VariableName=last_signal1  Interpolate=off  OutputAfterFinalValue=Holding final value
  Scope : Scope
      settings: ActiveDisplayYMinimum=-321.52156371284451  ActiveDisplayYMaximum=409.38065684966335
  Scope4 : Scope
      settings: ActiveDisplayYMinimum=-724.32967100373537  ActiveDisplayYMaximum=544.90361596398475
  Simulink-PS Converter : nesl_utility/Simulink-PS Converter  PhysicalDomain=network_engine_domain  SubClassName=ps_input  LeftPortType=input  RightPortType=output  PseudoPeriodic=off  Frequencies=[]  NoiseDistribution=none  NoiseParameters=[]  Unit=1  AffineConversion=off  FilteringAndDerivatives=provide  SimscapeFilterOrder=1  InputFilterTimeConstant=0.001  UdotUserProvided=0
  Simulink-PS Converter1 : nesl_utility/Simulink-PS Converter  PhysicalDomain=network_engine_domain  SubClassName=ps_input  LeftPortType=input  RightPortType=output  PseudoPeriodic=off  Frequencies=[]  NoiseDistribution=none  NoiseParameters=[]  Unit=1  AffineConversion=off  FilteringAndDerivatives=provide  SimscapeFilterOrder=1  InputFilterTimeConstant=0.001  UdotUserProvided=0
  "Wye-Connected Variable Load (lagging) " : ee_lib/Passive/RLC Assemblies/Wye-Connected Variable Load (lagging)  port_option=ee.enum.threePhasePort.composite  VRated=400 V  FRated=50 Hz  Pmin=1e3 W  Qmin=1e3 A*V  G_parasitic=1e-6 1/Ohm  I_specify=off  I_priority=None  I=[0, 0, 0] A  I_nominal_specify=off  I_nominal_value=1  I_nominal_unit=A  Phi_specify=off  Phi_priority=None  Phi=[0, 0, 0] Wb  Phi_nominal_specify=off  Phi_nominal_value=1  Phi_nominal_unit=Wb
  AC : PMIOPort  Side=Left
  Jord : PMIOPort  Port=2  Side=Left
  Jord fra solcelle : PMIOPort  Port=3  Side=Left
  Solcelle indfødning : PMIOPort  Port=4  Side=Left
  wires:
  Gain/1 -> Simulink-PS Converter1/1
  From Workspace/1 -> Gain/1
  Sat til sample time 0 for at være kontinuerlig/1 -> Simulink-PS Converter/1
  PS-Simulink Converter/1 -> Scope/1
  PS-Simulink Converter3/1 -> Scope4/1
  connections:
  Simulink-PS Converter1/RConn1 -- "Wye-Connected Variable Load (lagging) "/LConn2
  Simulink-PS Converter/RConn1 -- "Wye-Connected Variable Load (lagging) "/LConn1
  Current Sensor (Three-Phase)/RConn1 -- PS-Simulink Converter/LConn1
  Line Voltage Sensor (Three-Phase)/RConn1 -- PS-Simulink Converter3/LConn1
  "Wye-Connected Variable Load (lagging) "/RConn1 -- Jord fra solcelle/RConn1 -- Jord/RConn1
  Line Voltage Sensor (Three-Phase)/LConn1 -- Solcelle indfødning/RConn1 -- AC/RConn1 -- Current Sensor (Three-Phase)/LConn1
  Current Sensor (Three-Phase)/RConn2 -- "Wye-Connected Variable Load (lagging) "/LConn3

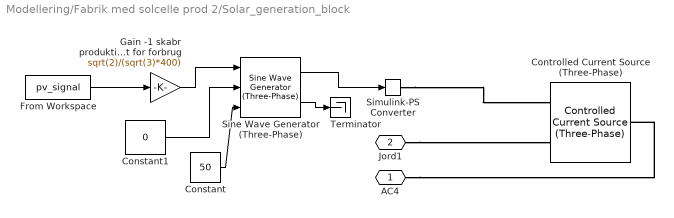
== system Modellering/Fabrik med solcelle prod 2/Solar_generation_block ==
  Constant : Constant  Value=50
  Constant1 : Constant  Value=0
  Controlled Current Source (Three-Phase) : ee_lib/Sources/Controlled Current Source (Three-Phase)  port_option=ee.enum.threePhasePort.composite  input_option=ee.enum.inputType.instantaneous  FRated=60 Hz  G_parasitic=1e-6 1/Ohm
  From Workspace : FromWorkspace  VariableName=pv_signal  Interpolate=off  OutputAfterFinalValue=Holding final value
  Gain -1 skabr produktion i stedet for forbrug : Gain  Gain=sqrt(2)/(sqrt(3)*400)
  Simulink-PS Converter : nesl_utility/Simulink-PS Converter  PhysicalDomain=network_engine_domain  SubClassName=ps_input  LeftPortType=input  RightPortType=output  PseudoPeriodic=off  Frequencies=[]  NoiseDistribution=none  NoiseParameters=[]  Unit=1  AffineConversion=off  FilteringAndDerivatives=provide  SimscapeFilterOrder=1  InputFilterTimeConstant=0.001  UdotUserProvided=0
  Sine Wave Generator (Three-Phase) : eeSinGeneratorThreePhase/Sine Wave Generator (Three-Phase)  Ts=0
      settings: LibrarySourceBlock=|
      | ee_sl_lib/General Control/Sine Wave Generator
      | (Three-Phase)
  Terminator : Terminator
  AC4 : PMIOPort  Side=Right
  Jord1 : PMIOPort  Port=2  Side=Left
  wires:
  Sine Wave Generator (Three-Phase)/2 -> Terminator/1
  Sine Wave Generator (Three-Phase)/1 -> Simulink-PS Converter/1
  Gain -1 skabr produktion i stedet for forbrug/1 -> Sine Wave Generator (Three-Phase)/1
  Constant1/1 -> Sine Wave Generator (Three-Phase)/2
  Constant/1 -> Sine Wave Generator (Three-Phase)/3
  From Workspace/1 -> Gain -1 skabr produktion i stedet for forbrug/1
  connections:
  Simulink-PS Converter/RConn1 -- Controlled Current Source (Three-Phase)/LConn1
  Jord1/RConn1 -- Controlled Current Source (Three-Phase)/LConn2
  AC4/RConn1 -- Controlled Current Source (Three-Phase)/RConn1

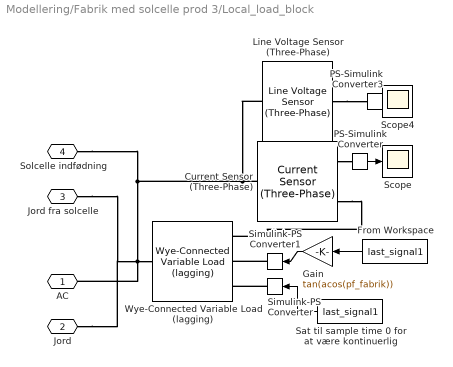
== system Modellering/Fabrik med solcelle prod 3/Local_load_block ==
  Current Sensor (Three-Phase) : ee_lib/Sensors & Transducers/Current Sensor (Three-Phase)  port_option=ee.enum.threePhasePort.composite
  From Workspace : FromWorkspace  VariableName=last_signal1
  Gain : Gain  Gain=tan(acos(pf_fabrik))
  Line Voltage Sensor (Three-Phase) : ee_lib/Sensors & Transducers/Line Voltage Sensor (Three-Phase)  port_option=ee.enum.threePhasePort.composite
  PS-Simulink Converter : nesl_utility/PS-Simulink Converter  PhysicalDomain=network_engine_domain  SubClassName=ps_output  LeftPortType=input  RightPortType=output  PseudoPeriodic=off  Frequencies=[]  VectorFormat=inherit  Unit=A  AffineConversion=off
  PS-Simulink Converter3 : nesl_utility/PS-Simulink Converter  PhysicalDomain=network_engine_domain  SubClassName=ps_output  LeftPortType=input  RightPortType=output  PseudoPeriodic=off  Frequencies=[]  VectorFormat=inherit  Unit=V  AffineConversion=off
  Sat til sample time 0 for at være kontinuerlig : FromWorkspace  VariableName=last_signal1  Interpolate=off  OutputAfterFinalValue=Holding final value
  Scope : Scope
      settings: ActiveDisplayYMinimum=-321.52156371284451  ActiveDisplayYMaximum=409.38065684966335
  Scope4 : Scope
      settings: ActiveDisplayYMinimum=-724.32967100373537  ActiveDisplayYMaximum=544.90361596398475
  Simulink-PS Converter : nesl_utility/Simulink-PS Converter  PhysicalDomain=network_engine_domain  SubClassName=ps_input  LeftPortType=input  RightPortType=output  PseudoPeriodic=off  Frequencies=[]  NoiseDistribution=none  NoiseParameters=[]  Unit=1  AffineConversion=off  FilteringAndDerivatives=provide  SimscapeFilterOrder=1  InputFilterTimeConstant=0.001  UdotUserProvided=0
  Simulink-PS Converter1 : nesl_utility/Simulink-PS Converter  PhysicalDomain=network_engine_domain  SubClassName=ps_input  LeftPortType=input  RightPortType=output  PseudoPeriodic=off  Frequencies=[]  NoiseDistribution=none  NoiseParameters=[]  Unit=1  AffineConversion=off  FilteringAndDerivatives=provide  SimscapeFilterOrder=1  InputFilterTimeConstant=0.001  UdotUserProvided=0
  "Wye-Connected Variable Load (lagging) " : ee_lib/Passive/RLC Assemblies/Wye-Connected Variable Load (lagging)  port_option=ee.enum.threePhasePort.composite  VRated=400 V  FRated=50 Hz  Pmin=1e3 W  Qmin=1e3 A*V  G_parasitic=1e-6 1/Ohm  I_specify=off  I_priority=None  I=[0, 0, 0] A  I_nominal_specify=off  I_nominal_value=1  I_nominal_unit=A  Phi_specify=off  Phi_priority=None  Phi=[0, 0, 0] Wb  Phi_nominal_specify=off  Phi_nominal_value=1  Phi_nominal_unit=Wb
  AC : PMIOPort  Side=Left
  Jord : PMIOPort  Port=2  Side=Left
  Jord fra solcelle : PMIOPort  Port=3  Side=Left
  Solcelle indfødning : PMIOPort  Port=4  Side=Left
  wires:
  Gain/1 -> Simulink-PS Converter1/1
  From Workspace/1 -> Gain/1
  Sat til sample time 0 for at være kontinuerlig/1 -> Simulink-PS Converter/1
  PS-Simulink Converter/1 -> Scope/1
  PS-Simulink Converter3/1 -> Scope4/1
  connections:
  Simulink-PS Converter1/RConn1 -- "Wye-Connected Variable Load (lagging) "/LConn2
  Simulink-PS Converter/RConn1 -- "Wye-Connected Variable Load (lagging) "/LConn1
  Current Sensor (Three-Phase)/RConn1 -- PS-Simulink Converter/LConn1
  Line Voltage Sensor (Three-Phase)/RConn1 -- PS-Simulink Converter3/LConn1
  "Wye-Connected Variable Load (lagging) "/RConn1 -- Jord fra solcelle/RConn1 -- Jord/RConn1
  Line Voltage Sensor (Three-Phase)/LConn1 -- Solcelle indfødning/RConn1 -- AC/RConn1 -- Current Sensor (Three-Phase)/LConn1
  Current Sensor (Three-Phase)/RConn2 -- "Wye-Connected Variable Load (lagging) "/LConn3

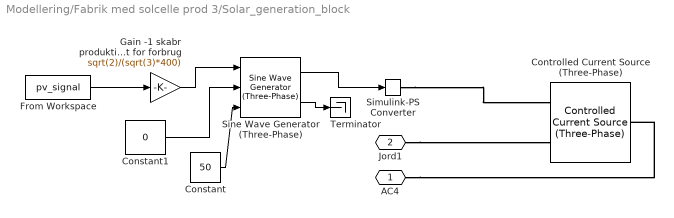
== system Modellering/Fabrik med solcelle prod 3/Solar_generation_block ==
  Constant : Constant  Value=50
  Constant1 : Constant  Value=0
  Controlled Current Source (Three-Phase) : ee_lib/Sources/Controlled Current Source (Three-Phase)  port_option=ee.enum.threePhasePort.composite  input_option=ee.enum.inputType.instantaneous  FRated=60 Hz  G_parasitic=1e-6 1/Ohm
  From Workspace : FromWorkspace  VariableName=pv_signal  Interpolate=off  OutputAfterFinalValue=Holding final value
  Gain -1 skabr produktion i stedet for forbrug : Gain  Gain=sqrt(2)/(sqrt(3)*400)
  Simulink-PS Converter : nesl_utility/Simulink-PS Converter  PhysicalDomain=network_engine_domain  SubClassName=ps_input  LeftPortType=input  RightPortType=output  PseudoPeriodic=off  Frequencies=[]  NoiseDistribution=none  NoiseParameters=[]  Unit=1  AffineConversion=off  FilteringAndDerivatives=provide  SimscapeFilterOrder=1  InputFilterTimeConstant=0.001  UdotUserProvided=0
  Sine Wave Generator (Three-Phase) : eeSinGeneratorThreePhase/Sine Wave Generator (Three-Phase)  Ts=0
      settings: LibrarySourceBlock=|
      | ee_sl_lib/General Control/Sine Wave Generator
      | (Three-Phase)
  Terminator : Terminator
  AC4 : PMIOPort  Side=Right
  Jord1 : PMIOPort  Port=2  Side=Left
  wires:
  Sine Wave Generator (Three-Phase)/2 -> Terminator/1
  Sine Wave Generator (Three-Phase)/1 -> Simulink-PS Converter/1
  Gain -1 skabr produktion i stedet for forbrug/1 -> Sine Wave Generator (Three-Phase)/1
  Constant1/1 -> Sine Wave Generator (Three-Phase)/2
  Constant/1 -> Sine Wave Generator (Three-Phase)/3
  From Workspace/1 -> Gain -1 skabr produktion i stedet for forbrug/1
  connections:
  Simulink-PS Converter/RConn1 -- Controlled Current Source (Three-Phase)/LConn1
  Jord1/RConn1 -- Controlled Current Source (Three-Phase)/LConn2
  AC4/RConn1 -- Controlled Current Source (Three-Phase)/RConn1
